simulink model "FCSMPC_IdealSDA"  (R2026a)
settings: Solver=FixedStepDiscrete  StopTime=inf  FixedStep=SimulinkTs
PreLoadFcn:
  | % Verzeichnis des Modells zum MATLAB-Pfad hinzufügen
  | modelDir = fileparts(get_param(bdroot, 'FileName'));
  | addpath(modelDir);
  | 
  | % Nur der Dateiname – kein Pfad!
  | set_param(bdroot, 'DataDictionary', 'FOC_params.sldd');
model workspace (MAT data in the model file):
  Np = Simulink.Parameter
  Np.Value = 5
  Np.Complexity = 'real'
  Np.Dimensions = [1 1]
  Np.DataType = 'double'
undefined symbols (not defined in the file or in its folder): dspblkCoreblockFVToolHelper, FCS, Filter, FOC, FOC_Control_Current_KIid, FOC_Control_Current_KIiq, FOC_Control_Current_KPid, FOC_Control_Current_KPiq, FOC_Control_Current_Krd, FOC_Control_Current_Krq, FOC_Control_Current_TclCur, FOC_Control_Current_Tnd, FOC_Control_Current_Tnq, FOC_Control_InverterVdc_V, FOC_Control_MotorImax_A, FOC_Control_MTPA_MTPV_nT_id_grid, FOC_Control_MTPA_MTPV_nT_iq_grid, FOC_Control_MTPA_MTPV_T_vec, FOC_Control_MTPA_MTPV_w_vec, FOC_Control_OpenLoop_Id_Ref_A, FOC_Control_OpenLoop_Iq_Ref_A, FOC_Control_OpenLoop_Ud_OpenLoop_V, FOC_Control_OpenLoop_Uq_OpenLoop_V, FOC_Control_RF_omegamech_rad_s, FOC_Control_RF_RateCurrent_A, FOC_Control_RF_RateTrq_Nm, FOC_Control_theta_mechOffsetFix, FOC_Control_theta_mechOffsetTime, FOC_Control_TorqueRef_Nm, FOC_Control_Umax_V, FOC_Flag_ClosedLoopControl, FOC_Flag_ControlStrategy, FOC_Flag_PWMEnable, FOC_Flag_ResetControl, FOC_Flag_TorqueControl, FOC_LUT_DQLimiter_DQ_LUTScaling, FOC_PWM_AZSPWMMethod, FOC_PWM_HybridMode, FOC_PWM_LB1, FOC_PWM_LB2, FOC_PWM_PWMManuel, FOC_PWM_RSPWMMethod, FOC_PWM_UB1, FOC_PWM_UB2, FOC_SampleTime_TsCur, gcbh, Plant, SimulinkTs
libraries: hdlsllib x2, autolibfluxpmsm x1, simulink x1
settings Model: DataDictionary=FOC_params.sldd  Creator=kara  LastModifiedBy=Cheng
settings DebuggingCC: ParameterPrecisionLossMsg=none
settings SimscapeCC: SimscapeNominalValues="[{\"value\":\"1\",\"unit\":\"A\"},{\"value\":\"1\",\"unit\":\"bar\"},{\"value\":\"1\",\"unit\":\"cm^2\"},{\"value\":\"1\",\"unit\":\"cm^3/s\"},{\"value\":\"1\",\"unit\":\"kJ/kg\"},{\"value\":\"1\",\"unit\":\"kW\"},{\"value\":\"1\",\"unit\":\"l\"},{\"value\":\"1\",\"unit\":\"N\"},{\"value\":\"1\",\"unit\":\"N*m\"},{\"value\":\"1\",\"unit\":\"V\"}]"  SimscapeLogType=none  SimscapeLogDataHistory=5000.0

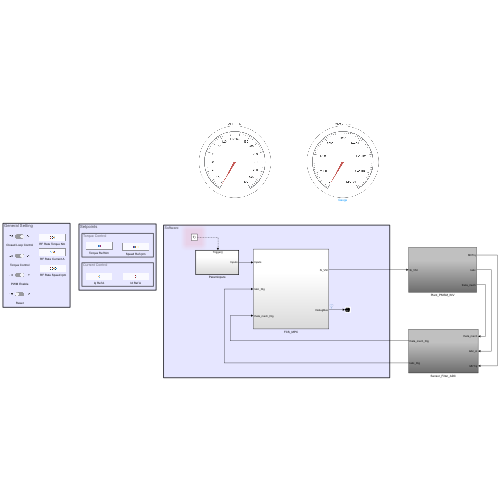
[thumbnail: Simulink's stored preview of the top-level diagram]
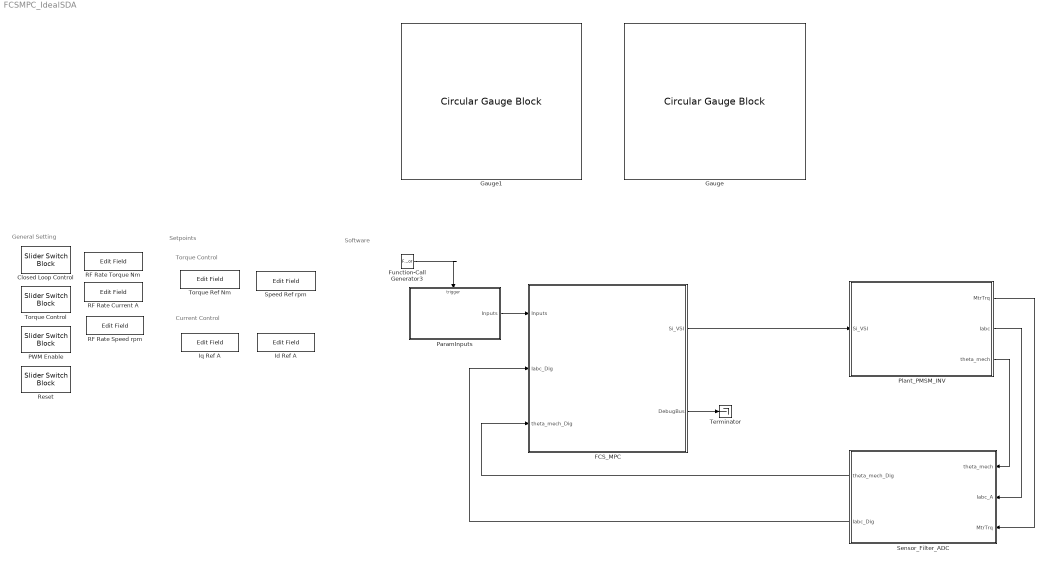
== system FCSMPC_IdealSDA ==
  note: Torque Control
  note: Software
  note: Current Control
  note: Setpoints
  note: General Setting
  Closed Loop Control : SliderSwitchBlock  LabelPosition=Hide
  FCS_MPC : Subsystem  VariantControl=AltPWM == 0
  Function-Call Generator3 : FunctionCallGenerator  SampleTime=FOC.SampleTime.TsSpeed
  Gauge : CircularGaugeBlock  ScaleMax=16000  FontColor=[0.0, 0.0, 0.0]
  Gauge1 : CircularGaugeBlock  ScaleMax=300  FontColor=[0.0, 0.0, 0.0]
  Id Ref A : EditField  LabelPosition=Hide  ShowInitialText=on  Alignment=Center
  Iq Ref A : EditField  LabelPosition=Hide  ShowInitialText=on  Alignment=Center
  PWM Enable : SliderSwitchBlock  LabelPosition=Hide
  ParamInputs : Subsystem
  Plant_PMSM_INV : Subsystem
  RF Rate Current A : EditField  LabelPosition=Hide  ShowInitialText=on  Alignment=Center
  RF Rate Speed rpm : EditField  LabelPosition=Hide  ShowInitialText=on  Alignment=Center
  RF Rate Torque Nm : EditField  LabelPosition=Hide  ShowInitialText=on  Alignment=Center
  Reset : SliderSwitchBlock  LabelPosition=Hide
  Sensor_Filter_ADC : Subsystem
  Speed Ref rpm : EditField  LabelPosition=Hide  ShowInitialText=on  Alignment=Center
  Terminator : Terminator
  Torque Control : SliderSwitchBlock  LabelPosition=Hide
  Torque Ref Nm : EditField  LabelPosition=Hide  ShowInitialText=on  Alignment=Center
  wires:
  ParamInputs/1(Inputs) -> FCS_MPC/1(Inputs)
  Function-Call Generator3/1 -> ParamInputs/Trigger
  Plant_PMSM_INV/2(Iabc) -> Sensor_Filter_ADC/2(Iabc_A)
  Plant_PMSM_INV/3(theta_mech) -> Sensor_Filter_ADC/1(theta_mech)
  FCS_MPC/1(Si_VSI) -> Plant_PMSM_INV/1(Si_VSI)
  Sensor_Filter_ADC/1(theta_mech_Dig) -> FCS_MPC/3(theta_mech_Dig)
  Plant_PMSM_INV/1(MtrTrq) -> Sensor_Filter_ADC/3(MtrTrq)
  Sensor_Filter_ADC/2(Iabc_Dig) -> FCS_MPC/2(Iabc_Dig)
  FCS_MPC/2(DebugBus) -> Terminator/1

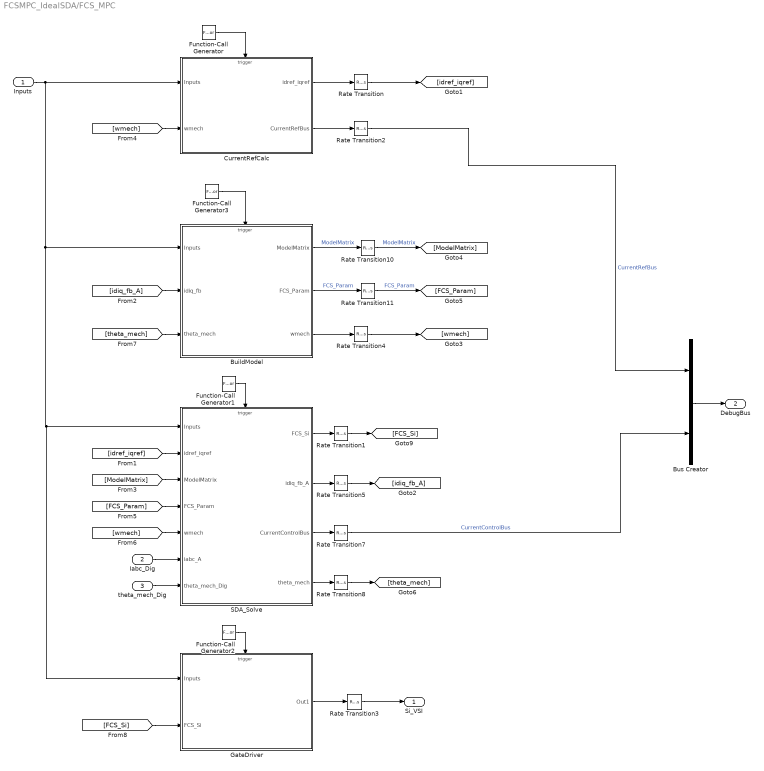
== system FCSMPC_IdealSDA/FCS_MPC ==
  Inputs : Inport
  Iabc_Dig : Inport  Port=2
  theta_mech_Dig : Inport  Port=3
  BuildModel : Subsystem
  Bus Creator : BusCreator  Inputs=2
  CurrentRefCalc : Subsystem
  Function-Call Generator : FunctionCallGenerator  SampleTime=FOC.SampleTime.TsSpeed
  Function-Call Generator1 : FunctionCallGenerator  SampleTime=FCS.Ts_SDA
  Function-Call Generator2 : FunctionCallGenerator  SampleTime=FOC.SampleTime.BSW.DeadTimeSample
  Function-Call Generator3 : FunctionCallGenerator  SampleTime=FCS.Ts_BuildModel
  GateDriver : Subsystem  TreatAsAtomicUnit=on
  Rate Transition{,1..5,7..8,10..11} (10 alike) : RateTransition  Deterministic=off
  SDA_Solve : Subsystem
  Si_VSI : Outport
  DebugBus : Outport  Port=2
  wires:
  Function-Call Generator/1 -> CurrentRefCalc/Trigger
  Function-Call Generator3/1 -> BuildModel/Trigger
  [wmech] -> CurrentRefCalc/2(wmech)
  CurrentRefCalc/1(idref_iqref) -> Rate Transition/1
  [idref_iqref] -> SDA_Solve/2(idref_iqref)
  Inputs/1 -> CurrentRefCalc/1(Inputs), GateDriver/1(Inputs), SDA_Solve/1(Inputs), BuildModel/1(Inputs)
  BuildModel/3(wmech) -> Rate Transition4/1
  CurrentRefCalc/2(CurrentRefBus) -> Rate Transition2/1
  Bus Creator/1 -> DebugBus/1
  Rate Transition/1 -> [idref_iqref]
  Rate Transition4/1 -> [wmech]
  Rate Transition2/1 -> Bus Creator/1  "CurrentRefBus"
  Rate Transition3/1 -> Si_VSI/1
  Function-Call Generator1/1 -> SDA_Solve/Trigger
  Iabc_Dig/1 -> SDA_Solve/6(iabc_A)
  SDA_Solve/2(idiq_fb_A) -> Rate Transition5/1
  Rate Transition5/1 -> [idiq_fb_A]
  [idiq_fb_A] -> BuildModel/2(idiq_fb)
  theta_mech_Dig/1 -> SDA_Solve/7(theta_mech_Dig)
  BuildModel/1(ModelMatrix) -> Rate Transition10/1  "ModelMatrix"
  BuildModel/2(FCS_Param) -> Rate Transition11/1  "FCS_Param"
  [ModelMatrix] -> SDA_Solve/3(ModelMatrix)
  [FCS_Param] -> SDA_Solve/4(FCS_Param)
  [wmech] -> SDA_Solve/5(wmech)
  SDA_Solve/3(CurrentControlBus) -> Rate Transition7/1
  Rate Transition7/1 -> Bus Creator/2  "CurrentControlBus"
  SDA_Solve/4(theta_mech) -> Rate Transition8/1
  Rate Transition8/1 -> [theta_mech]
  [theta_mech] -> BuildModel/3(theta_mech)
  Rate Transition11/1 -> [FCS_Param]  "FCS_Param"
  Rate Transition10/1 -> [ModelMatrix]  "ModelMatrix"
  Function-Call Generator2/1 -> GateDriver/Trigger
  GateDriver/1(Out1) -> Rate Transition3/1
  SDA_Solve/1(FCS_Si) -> Rate Transition1/1
  Rate Transition1/1 -> [FCS_Si]
  [FCS_Si] -> GateDriver/2(FCS_Si)

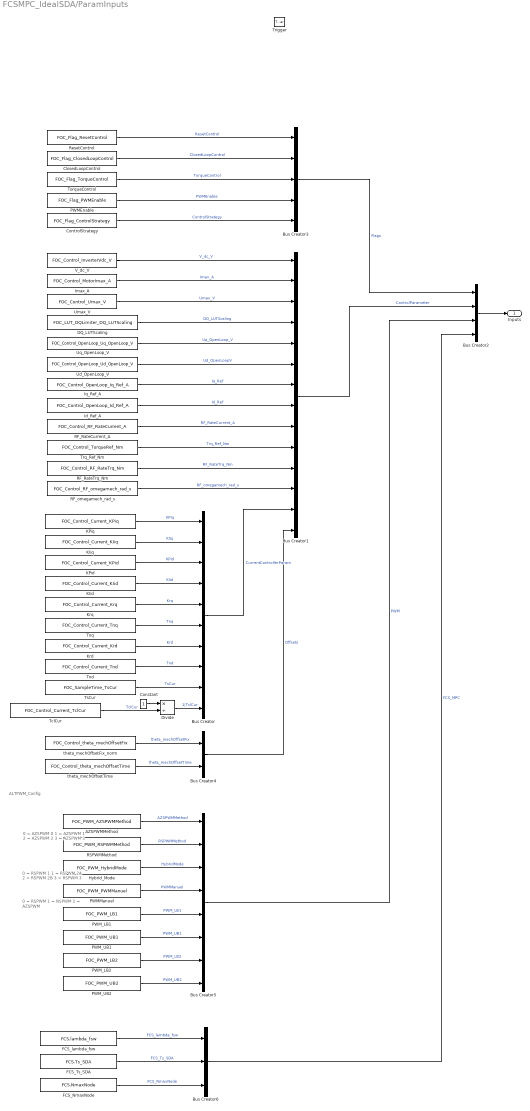
== system FCSMPC_IdealSDA/ParamInputs ==
  note: ALTPWM_Config
  note: 0 = RSPWM 1
      | 1 = RSPWM 2A
      | 2 = RSPWM 2B
      | 3 = RSPWM 3
  note: 0 = AZSPWM 0
      | 1 = AZSPWM 1
      | 2 = AZSPWM 2
      | 3 = AZSPWM 3
  note: 0 = RSPWM
      | 1 = NSPWM
      | 2 = AZSPWM
  Trigger : TriggerPort  TriggerType=function-call  VariantControl=(inherit)  SampleTimeType=periodic  SampleTime=FOC.SampleTime.TsSpeed  PortDimensions=1
  AZSPWMMethod : Constant  Value=FOC_PWM_AZSPWMMethod
  Bus Creator : BusCreator  Inputs=10
  Bus Creator1 : BusCreator  Inputs=14
  Bus Creator2 : BusCreator  Inputs=4
  Bus Creator3 : BusCreator  Inputs=5
  Bus Creator4 : BusCreator  Inputs=2
  Bus Creator5 : BusCreator  Inputs=8
  Bus Creator6 : BusCreator  Inputs=3
  ClosedLoopControl : Constant  Value=FOC_Flag_ClosedLoopControl
  Constant : Constant  OutDataTypeStr=SIScaling  SampleTime=-1
  ControlStrategy : Constant  Value=FOC_Flag_ControlStrategy
  DQ_LUTScaling : Constant  Value=FOC_LUT_DQLimiter_DQ_LUTScaling
  Divide : Product  Inputs=*/  OutDataTypeStr=SIScaling
  FCS_NmaxNode : Constant  Value=FCS.NmaxNode
  FCS_Ts_SDA : Constant  Value=FCS.Ts_SDA
  FCS_lambda_fsw : Constant  Value=FCS.lambda_fsw
  Hybrid_Mode : Constant  Value=FOC_PWM_HybridMode
  Id_Ref_A : Constant  Value=FOC_Control_OpenLoop_Id_Ref_A
  Imax_A : Constant  Value=FOC_Control_MotorImax_A
  Iq_Ref_A : Constant  Value=FOC_Control_OpenLoop_Iq_Ref_A
  KIid : Constant  Value=FOC_Control_Current_KIid
  KIiq : Constant  Value=FOC_Control_Current_KIiq
  KPid : Constant  Value=FOC_Control_Current_KPid
  KPiq : Constant  Value=FOC_Control_Current_KPiq
  Krd : Constant  Value=FOC_Control_Current_Krd
  Krq : Constant  Value=FOC_Control_Current_Krq
  PWMEnable : Constant  Value=FOC_Flag_PWMEnable
  PWMManuel : Constant  Value=FOC_PWM_PWMManuel
  PWM_LB1 : Constant  Value=FOC_PWM_LB1
  PWM_LB2 : Constant  Value=FOC_PWM_LB2
  PWM_UB1 : Constant  Value=FOC_PWM_UB1
  PWM_UB2 : Constant  Value=FOC_PWM_UB2
  RF_RateCurrent_A : Constant  Value=FOC_Control_RF_RateCurrent_A
  RF_RateTrq_Nm : Constant  Value=FOC_Control_RF_RateTrq_Nm
  RF_omegamech_rad_s : Constant  Value=FOC_Control_RF_omegamech_rad_s
  RSPWMMethod : Constant  Value=FOC_PWM_RSPWMMethod
  ResetControl : Constant  Value=FOC_Flag_ResetControl
  TclCur : Constant  Value=FOC_Control_Current_TclCur
  Tnd : Constant  Value=FOC_Control_Current_Tnd
  Tnq : Constant  Value=FOC_Control_Current_Tnq
  TorqueControl : Constant  Value=FOC_Flag_TorqueControl
  Trq_Ref_Nm : Constant  Value=FOC_Control_TorqueRef_Nm
  TsCur : Constant  Value=FOC_SampleTime_TsCur
  Ud_OpenLoop_V : Constant  Value=FOC_Control_OpenLoop_Ud_OpenLoop_V
  Umax_V : Constant  Value=FOC_Control_Umax_V
  Uq_OpenLoop_V : Constant  Value=FOC_Control_OpenLoop_Uq_OpenLoop_V
  V_dc_V : Constant  Value=FOC_Control_InverterVdc_V
  theta_mechOffsetFix_norm : Constant  Value=FOC_Control_theta_mechOffsetFix
  theta_mechOffsetTime : Constant  Value=FOC_Control_theta_mechOffsetTime
  Inputs : Outport
  wires:
  Bus Creator2/1 -> Inputs/1
  ClosedLoopControl/1 -> Bus Creator3/2  "ClosedLoopControl"
  TorqueControl/1 -> Bus Creator3/3  "TorqueControl"
  PWMEnable/1 -> Bus Creator3/4  "PWMEnable"
  Bus Creator3/1 -> Bus Creator2/1  "Flags"
  ResetControl/1 -> Bus Creator3/1  "ResetControl"
  ControlStrategy/1 -> Bus Creator3/5  "ControlStrategy"
  Ud_OpenLoop_V/1 -> Bus Creator1/6  "Ud_OpenLoopV"
  Uq_OpenLoop_V/1 -> Bus Creator1/5  "Uq_OpenLoop_V"
  DQ_LUTScaling/1 -> Bus Creator1/4  "DQ_LUTScaling"
  Umax_V/1 -> Bus Creator1/3  "Umax_V"
  Bus Creator1/1 -> Bus Creator2/2  "ControlParameter"
  Iq_Ref_A/1 -> Bus Creator1/7  "Iq_Ref"
  Id_Ref_A/1 -> Bus Creator1/8  "Id_Ref"
  Imax_A/1 -> Bus Creator1/2  "Imax_A"
  RF_RateTrq_Nm/1 -> Bus Creator1/11  "RF_RateTrq_Nm"
  Trq_Ref_Nm/1 -> Bus Creator1/10  "Trq_Ref_Nm"
  RF_RateCurrent_A/1 -> Bus Creator1/9  "RF_RateCurrent_A"
  Bus Creator/1 -> Bus Creator1/13  "CurrentControllerParam"
  V_dc_V/1 -> Bus Creator1/1  "V_dc_V"
  RF_omegamech_rad_s/1 -> Bus Creator1/12  "RF_omegamech_rad_s"
  theta_mechOffsetFix_norm/1 -> Bus Creator4/1  "theta_mechOffsetFix"
  theta_mechOffsetTime/1 -> Bus Creator4/2  "theta_mechOffsetTime"
  Bus Creator4/1 -> Bus Creator1/14  "Offsets"
  Bus Creator5/1 -> Bus Creator2/3  "PWM"
  PWM_UB1/1 -> Bus Creator5/6  "PWM_UB1"
  PWM_LB2/1 -> Bus Creator5/7  "PWM_LB2"
  AZSPWMMethod/1 -> Bus Creator5/1  "AZSPWMMethod"
  RSPWMMethod/1 -> Bus Creator5/2  "RSPWMMethod"
  PWM_LB1/1 -> Bus Creator5/5  "PWM_LB1"
  PWM_UB2/1 -> Bus Creator5/8  "PWM_UB2"
  Hybrid_Mode/1 -> Bus Creator5/3  "HybridMode"
  PWMManuel/1 -> Bus Creator5/4  "PWMManuel"
  TsCur/1 -> Bus Creator/9  "TsCur"
  KIiq/1 -> Bus Creator/2  "KIiq"
  Tnq/1 -> Bus Creator/6  "Tnq"
  Krd/1 -> Bus Creator/7  "Krd"
  KPid/1 -> Bus Creator/3  "KPid"
  Krq/1 -> Bus Creator/5  "Krq"
  Tnd/1 -> Bus Creator/8  "Tnd"
  KIid/1 -> Bus Creator/4  "KIid"
  KPiq/1 -> Bus Creator/1  "KPiq"
  TclCur/1 -> Divide/2  "TclCur"
  Divide/1 -> Bus Creator/10  "1|TclCur"
  Constant/1 -> Divide/1
  FCS_Ts_SDA/1 -> Bus Creator6/2  "FCS_Ts_SDA"
  FCS_lambda_fsw/1 -> Bus Creator6/1  "FCS_lambda_fsw"
  Bus Creator6/1 -> Bus Creator2/4  "FCS_MPC"
  FCS_NmaxNode/1 -> Bus Creator6/3  "FCS_NmaxNode"

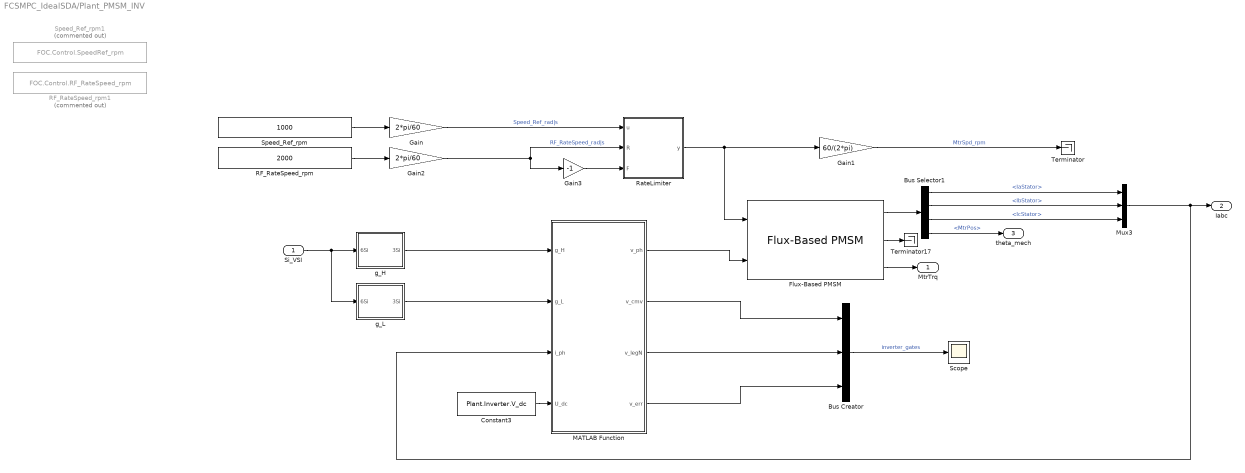
== system FCSMPC_IdealSDA/Plant_PMSM_INV ==
  Si_VSI : Inport
  Bus Creator : BusCreator  Inputs=3
  Bus Selector1 : BusSelector  OutputSignals=IaStator,IbStator,IcStator,MtrPos
  Constant3 : Constant  Value=Plant.Inverter.V_dc  SampleTime=-1
  Flux-Based PMSM : autolibfluxpmsm/Flux-Based PMSM  sim_type=Discrete  Ts=SimulinkTs  port_config=Speed  enable_hdl=off  flux_d=Plant.Fluxd_vec  n1=2  flux_q=Plant.Fluxq_vec  n2=2  id=Plant.FluxdFluxq_Id_grid'  iq=Plant.FluxdFluxq_Iq_grid'  preExtrapFlag=off  u1max=0.22457  u1min=-0.22607  u2max=0.42959  u2min=-0.4296  Rs=Plant.Motor.Rs  P=Plant.Motor.p  fluxdq0=[0 0]  theta_init=0  omega_init=0  mechanical=[0.0027, 4.924e-4, 0]  RefBlkName='autolibfluxpmsm/Flux-Based PMSM'  intPrec=23
      settings: LibrarySourceBlock=autolibemachines/Flux-Based PMSM
  Gain : Gain  Gain=2*pi/60
  Gain1 : Gain  Gain=60/(2*pi)
  Gain2 : Gain  Gain=2*pi/60
  Gain3 : Gain  Gain=-1
  MATLAB Function : MATLAB Function  TreatAsAtomicUnit=on
  Mux3 : Mux  Inputs=3
  RF_RateSpeed_rpm : Constant  Value=2000
  RF_RateSpeed_rpm1 : Constant  Commented=on  Value=FOC.Control.RF_RateSpeed_rpm
  RateLimiter : Stateflow chart  TreatAsAtomicUnit=on
  Scope : Scope
  Speed_Ref_rpm : Constant  Value=1000
  Speed_Ref_rpm1 : Constant  Commented=on  Value=FOC.Control.SpeedRef_rpm
  Terminator : Terminator
  Terminator17 : Terminator
  g_H : Subsystem
  g_L : Subsystem
  MtrTrq : Outport
  Iabc : Outport  Port=2
  theta_mech : Outport  Port=3
  wires:
  RateLimiter/1(y) -> Flux-Based PMSM/1, Gain1/1
  g_H/1(3Si) -> MATLAB Function/1(g_H)
  Bus Selector1/2 -> Mux3/2  "<IbStator>"
  Si_VSI/1 -> g_L/1(6Si), g_H/1(6Si)
  Bus Selector1/1 -> Mux3/1  "<IaStator>"
  Constant3/1 -> MATLAB Function/4(U_dc)
  Flux-Based PMSM/2 -> Terminator17/1
  Flux-Based PMSM/1 -> Bus Selector1/1
  Bus Selector1/3 -> Mux3/3  "<IcStator>"
  Gain1/1 -> Terminator/1  "MtrSpd_rpm"
  Flux-Based PMSM/3 -> MtrTrq/1
  Mux3/1 -> MATLAB Function/3(i_ph), Iabc/1
  Bus Selector1/4 -> theta_mech/1  "<MtrPos>"
  Gain3/1 -> RateLimiter/3(F)
  RF_RateSpeed_rpm/1 -> Gain2/1
  Speed_Ref_rpm/1 -> Gain/1
  Gain/1 -> RateLimiter/1(u)  "Speed_Ref_rad|s"
  Gain2/1 -> RateLimiter/2(R), Gain3/1  "RF_RateSpeed_rad|s"
  g_L/1(3Si) -> MATLAB Function/2(g_L)
  MATLAB Function/1(v_ph) -> Flux-Based PMSM/2
  MATLAB Function/2(v_cmv) -> Bus Creator/1
  MATLAB Function/4(v_err) -> Bus Creator/3
  MATLAB Function/3(v_legN) -> Bus Creator/2
  Bus Creator/1 -> Scope/1  "inverter_gates"

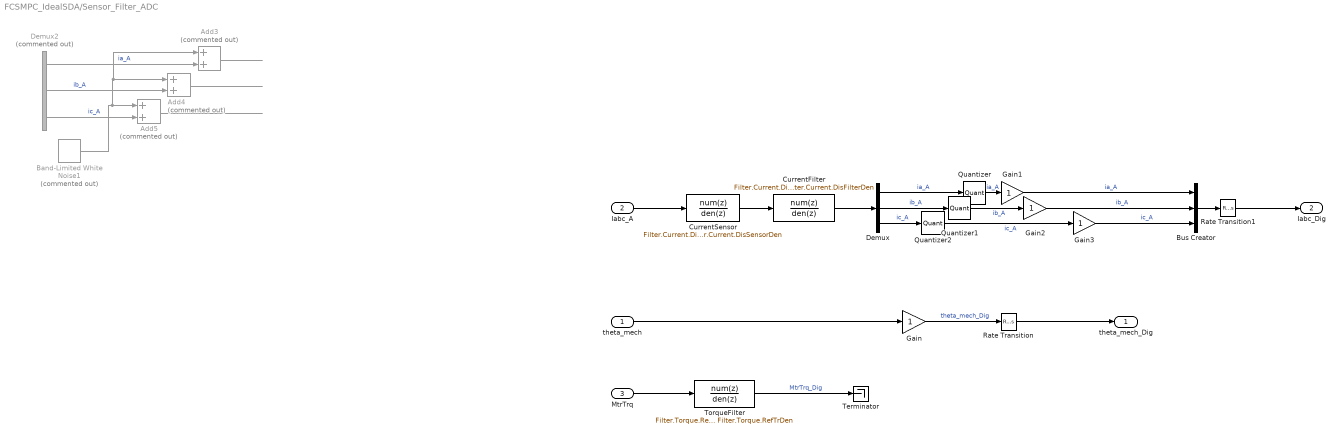
== system FCSMPC_IdealSDA/Sensor_Filter_ADC ==
  theta_mech : Inport
  Iabc_A : Inport  Port=2
  MtrTrq : Inport  Port=3
  Add3 : Sum  Commented=on
  Add4 : Sum  Commented=on
  Add5 : Sum  Commented=on
  Band-Limited White Noise1 : simulink/Sources/Band-Limited White Noise  Commented=on  Cov=[0.00001]  Ts=SimulinkTs  seed=[23341]
  Bus Creator : BusCreator  Inputs=3
  CurrentFilter : DiscreteTransferFcn  Numerator=Filter.Current.DisFilterNum  Denominator=Filter.Current.DisFilterDen
  CurrentSensor : DiscreteTransferFcn  LoadFcn=dspblkCoreblockFVToolHelper(gcbh,'load');  Numerator=Filter.Current.DisSensorNum  Denominator=Filter.Current.DisSensorDen
      settings: CopyFcn=dspblkCoreblockFVToolHelper(gcbh,'copy');  DeleteFcn=dspblkCoreblockFVToolHelper(gcbh,'close');  ModelCloseFcn=dspblkCoreblockFVToolHelper(gcbh,'close');  PreSaveFcn=dspblkCoreblockFVToolHelper(gcbh,'presave');  PostSaveFcn=dspblkCoreblockFVToolHelper(gcbh,'postsave');  CloseFcn=dspblkCoreblockFVToolHelper(gcbh,'close');
  Demux : Demux  Outputs=3
  Demux2 : Demux  Commented=on  Outputs=3
  Gain : Gain  OutDataTypeStr=HighScaling
  Gain1 : Gain  OutDataTypeStr=SIScaling
  Gain2 : Gain  OutDataTypeStr=SIScaling
  Gain3 : Gain  OutDataTypeStr=SIScaling
  Quantizer : Quantizer  QuantizationInterval=(10/32767)*264.04
  Quantizer1 : Quantizer  QuantizationInterval=(10/32767)*264.04
  Quantizer2 : Quantizer  QuantizationInterval=(10/32767)*264.04
  Rate Transition : RateTransition  Deterministic=off
  Rate Transition1 : RateTransition  Deterministic=off
  Terminator : Terminator
  TorqueFilter : DiscreteTransferFcn  Numerator=Filter.Torque.RefTrNum  Denominator=Filter.Torque.RefTrDen
  theta_mech_Dig : Outport
  Iabc_Dig : Outport  Port=2
  wires:
  MtrTrq/1 -> TorqueFilter/1
  CurrentSensor/1 -> CurrentFilter/1
  CurrentFilter/1 -> Demux/1
  TorqueFilter/1 -> Terminator/1  "MtrTrq_Dig"
  Demux/2 -> Quantizer1/1  "ib_A"
  Demux/3 -> Quantizer2/1  "ic_A"
  Demux/1 -> Quantizer/1  "ia_A"
  Bus Creator/1 -> Rate Transition1/1
  Gain/1 -> Rate Transition/1  "theta_mech_Dig"
  Gain1/1 -> Bus Creator/1  "ia_A"
  Gain2/1 -> Bus Creator/2  "ib_A"
  Gain3/1 -> Bus Creator/3  "ic_A"
  Rate Transition/1 -> theta_mech_Dig/1
  Rate Transition1/1 -> Iabc_Dig/1
  theta_mech/1 -> Gain/1
  Quantizer/1 -> Gain1/1  "ia_A"
  Quantizer1/1 -> Gain2/1  "ib_A"
  Quantizer2/1 -> Gain3/1  "ic_A"
  Iabc_A/1 -> CurrentSensor/1
  Demux2/1 -> Add3/2  "ia_A"
  Demux2/2 -> Add4/2  "ib_A"
  Demux2/3 -> Add5/2  "ic_A"
  Add5/1 -> ?
  Add4/1 -> ?
  Add3/1 -> ?
  ? -> Demux2/1
  Band-Limited White Noise1/1 -> Add5/1, Add4/1, Add3/1

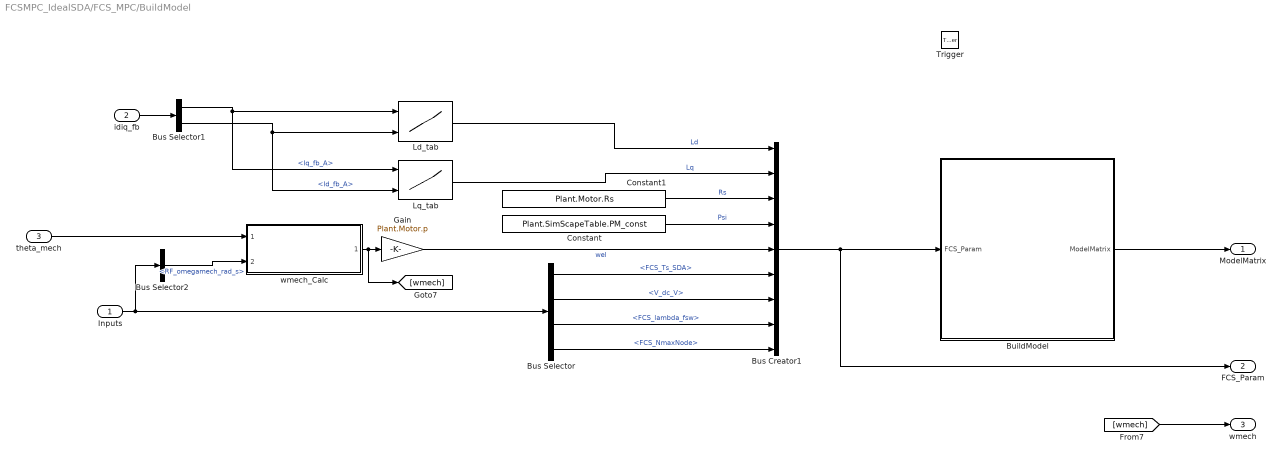
== system FCSMPC_IdealSDA/FCS_MPC/BuildModel ==
  Inputs : Inport
  idiq_fb : Inport  Port=2
  theta_mech : Inport  Port=3
  Trigger : TriggerPort  TriggerType=function-call  VariantControl=(inherit)  PropagateVarSize=Only when enabling  SampleTimeType=periodic  SampleTime=FCS.Ts_BuildModel  InitialTriggerSignalState=positive  PortDimensions=1
  BuildModel : Subsystem
  Bus Creator1 : BusCreator  Inputs=9
  Bus Selector : BusSelector  OutputSignals=FCS_MPC.FCS_Ts_SDA,ControlParameter.V_dc_V,FCS_MPC.FCS_lambda_fsw,FCS_MPC.FCS_NmaxNode
  Bus Selector1 : BusSelector  OutputSignals=Iq_fb_A,Id_fb_A
  Bus Selector2 : BusSelector  OutputSignals=ControlParameter.RF_omegamech_rad_s
  Constant : Constant  Value=Plant.SimScapeTable.PM_const  OutDataTypeStr=PWMGenSacling  SampleTime=-1
  Constant1 : Constant  Value=Plant.Motor.Rs  OutDataTypeStr=PWMGenSacling  SampleTime=-1
  Gain : Gain  Gain=Plant.Motor.p  OutDataTypeStr=RoughScaling
  Ld_tab : Lookup_n-D  BreakpointsForDimension1=Plant.SimScapeTable.iQ_vec  BreakpointsForDimension2=Plant.SimScapeTable.iD_vec  Table=Plant.SimScapeTable.Ld_tab'  ExtrapMethod=Clip  InternalRulePriority=Speed  RndMeth=Simplest
      settings: InputPortMap=u0,u1
  Lq_tab : Lookup_n-D  BreakpointsForDimension1=Plant.SimScapeTable.iQ_vec  BreakpointsForDimension2=Plant.SimScapeTable.iD_vec  Table=Plant.SimScapeTable.Lq_tab'  ExtrapMethod=Clip  InternalRulePriority=Speed  RndMeth=Simplest
      settings: InputPortMap=u0,u1
  wmech_Calc : Subsystem  ReferencedSubsystem=wmech_Calc
  ModelMatrix : Outport
  FCS_Param : Outport  Port=2
  wmech : Outport  Port=3
  wires:
  Ld_tab/1 -> Bus Creator1/1  "Ld"
  Lq_tab/1 -> Bus Creator1/2  "Lq"
  Constant/1 -> Bus Creator1/4  "Psi"
  Bus Selector/1 -> Bus Creator1/6  "<FCS_Ts_SDA>"
  Bus Selector/2 -> Bus Creator1/7  "<V_dc_V>"
  Bus Creator1/1 -> FCS_Param/1, BuildModel/1(FCS_Param)
  BuildModel/1(ModelMatrix) -> ModelMatrix/1
  Gain/1 -> Bus Creator1/5  "wel"
  Bus Selector/4 -> Bus Creator1/9  "<FCS_NmaxNode>"
  Bus Selector/3 -> Bus Creator1/8  "<FCS_lambda_fsw>"
  idiq_fb/1 -> Bus Selector1/1
  Bus Selector1/2 -> Lq_tab/2, Ld_tab/2  "<Id_fb_A>"
  Bus Selector1/1 -> Lq_tab/1, Ld_tab/1  "<Iq_fb_A>"
  Constant1/1 -> Bus Creator1/3  "Rs"
  theta_mech/1 -> wmech_Calc/1
  Bus Selector2/1 -> wmech_Calc/2  "<RF_omegamech_rad_s>"
  Inputs/1 -> Bus Selector/1, Bus Selector2/1
  [wmech] -> wmech/1
  wmech_Calc/1 -> [wmech], Gain/1

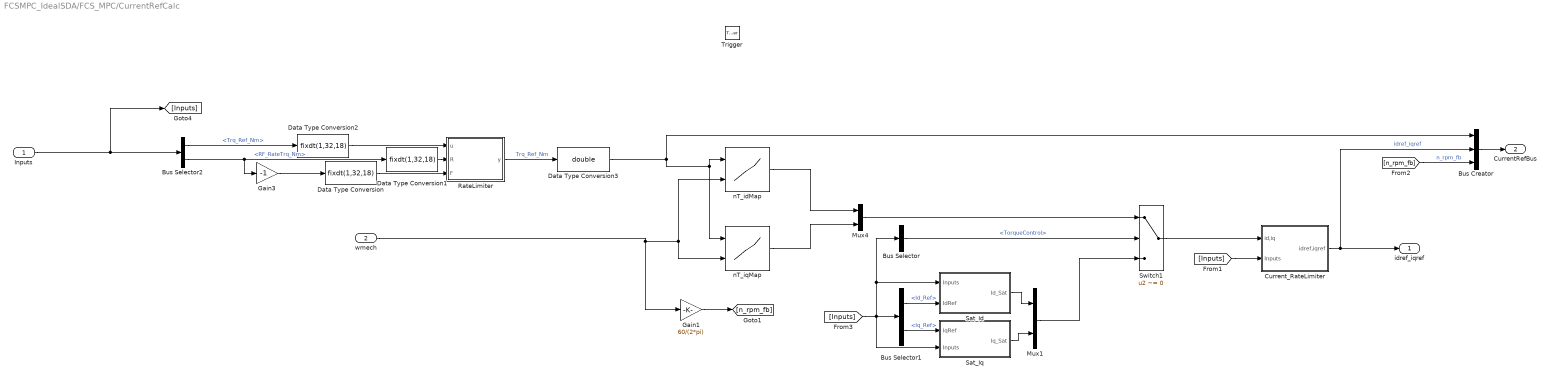
== system FCSMPC_IdealSDA/FCS_MPC/CurrentRefCalc ==
  Inputs : Inport
  wmech : Inport  Port=2
  Trigger : TriggerPort  TriggerType=function-call  VariantControl=(inherit)  PropagateVarSize=Only when enabling  SampleTimeType=periodic  SampleTime=FOC.SampleTime.TsSpeed  InitialTriggerSignalState=positive  PortDimensions=1
  Bus Creator : BusCreator  Inputs=3
  Bus Selector : BusSelector  OutputSignals=Flags.TorqueControl
  Bus Selector1 : BusSelector  OutputSignals=ControlParameter.Id_Ref,ControlParameter.Iq_Ref
  Bus Selector2 : BusSelector  OutputSignals=ControlParameter.Trq_Ref_Nm,ControlParameter.RF_RateTrq_Nm
  Current_RateLimiter : Subsystem
  Data Type Conversion : DataTypeConversion  OutDataTypeStr=fixdt(1,32,18)  SaturateOnIntegerOverflow=off  RndMeth=Floor
  Data Type Conversion1 : DataTypeConversion  OutDataTypeStr=fixdt(1,32,18)  SaturateOnIntegerOverflow=off  RndMeth=Floor
  Data Type Conversion2 : DataTypeConversion  OutDataTypeStr=fixdt(1,32,18)  SaturateOnIntegerOverflow=off  RndMeth=Floor
  Data Type Conversion3 : DataTypeConversion  OutDataTypeStr=double  SaturateOnIntegerOverflow=off  RndMeth=Floor
  Gain1 : Gain  Gain=60/(2*pi)  OutDataTypeStr=SIScaling
  Gain3 : Gain  Gain=-1  OutDataTypeStr=SIScaling
  Mux1 : Mux  Inputs=2
  Mux4 : Mux  Inputs=2
  RateLimiter : Stateflow chart  TreatAsAtomicUnit=on
  Sat_Id : Subsystem
  Sat_Iq : Subsystem
  Switch1 : Switch  Criteria=u2 ~= 0  OutDataTypeStr=SIScaling  SaturateOnIntegerOverflow=off  InputSameDT=off
  nT_idMap : Lookup_n-D  BreakpointsForDimension1=FOC_Control_MTPA_MTPV_T_vec  BreakpointsForDimension2=FOC_Control_MTPA_MTPV_w_vec  Table=FOC_Control_MTPA_MTPV_nT_id_grid  ExtrapMethod=Clip  InternalRulePriority=Speed  RndMeth=Simplest
      settings: InputPortMap=u0,u1
  nT_iqMap : Lookup_n-D  BreakpointsForDimension1=FOC_Control_MTPA_MTPV_T_vec  BreakpointsForDimension2=FOC_Control_MTPA_MTPV_w_vec  Table=FOC_Control_MTPA_MTPV_nT_iq_grid  ExtrapMethod=Clip  InternalRulePriority=Speed  RndMeth=Simplest
      settings: InputPortMap=u0,u1
  idref_iqref : Outport
  CurrentRefBus : Outport  Port=2
  wires:
  Bus Selector2/2 -> Data Type Conversion1/1, Gain3/1  "<RF_RateTrq_Nm>"
  Gain3/1 -> Data Type Conversion/1
  RateLimiter/1(y) -> Data Type Conversion3/1  "Trq_Ref_Nm"
  nT_iqMap/1 -> Mux4/2
  nT_idMap/1 -> Mux4/1
  Mux4/1 -> Switch1/1
  Bus Selector/1 -> Switch1/2  "<TorqueControl>"
  Bus Selector1/1 -> Sat_Id/2(IdRef)  "<Id_Ref>"
  Bus Selector1/2 -> Sat_Iq/1(IqRef)  "<Iq_Ref>"
  Mux1/1 -> Switch1/3
  Sat_Id/1(Id_Sat) -> Mux1/1
  Sat_Iq/1(Iq_Sat) -> Mux1/2
  Inputs/1 -> Bus Selector2/1, [Inputs]
  [Inputs] -> Sat_Iq/2(Inputs), Bus Selector/1, Sat_Id/1(Inputs), Bus Selector1/1
  Bus Selector2/1 -> Data Type Conversion2/1  "<Trq_Ref_Nm>"
  Switch1/1 -> Current_RateLimiter/1(id,iq)
  [Inputs] -> Current_RateLimiter/2(Inputs)
  Current_RateLimiter/1(idref,iqref) -> idref_iqref/1, Bus Creator/2  "idref_iqref"
  Bus Creator/1 -> CurrentRefBus/1
  [n_rpm_fb] -> Bus Creator/3  "n_rpm_fb"
  wmech/1 -> Gain1/1, nT_iqMap/2, nT_idMap/2
  Gain1/1 -> [n_rpm_fb]
  Data Type Conversion/1 -> RateLimiter/3(F)
  Data Type Conversion1/1 -> RateLimiter/2(R)
  Data Type Conversion2/1 -> RateLimiter/1(u)
  Data Type Conversion3/1 -> nT_iqMap/1, nT_idMap/1, Bus Creator/1

== system FCSMPC_IdealSDA/FCS_MPC/GateDriver ==
  Inputs : Inport
  FCS_Si : Inport  Port=2
  Trigger : TriggerPort  TriggerType=function-call  VariantControl=(inherit)  SampleTimeType=periodic  SampleTime=FOC.SampleTime.BSW.DeadTimeSample
  Bus Selector : BusSelector  OutputSignals=Flags.PWMEnable
  Constant4 : Constant  Value=[0 0 0 0 0 0]  OutDataTypeStr=uint8  SampleTime=-1
  GateDriver : Subsystem  ReferencedSubsystem=GateDriver  DeadTime=FOC.SampleTime.BSW.DeadTime  DeadTimeSample=FOC.SampleTime.BSW.DeadTimeSample
  Switch1 : Switch  Criteria=u2 ~= 0  SaturateOnIntegerOverflow=off  InputSameDT=off
  Out1 : Outport
  wires:
  FCS_Si/1 -> GateDriver/1
  GateDriver/1 -> Switch1/1
  Constant4/1 -> Switch1/3
  Switch1/1 -> Out1/1
  Inputs/1 -> Bus Selector/1
  Bus Selector/1 -> Switch1/2  "<PWMEnable>"

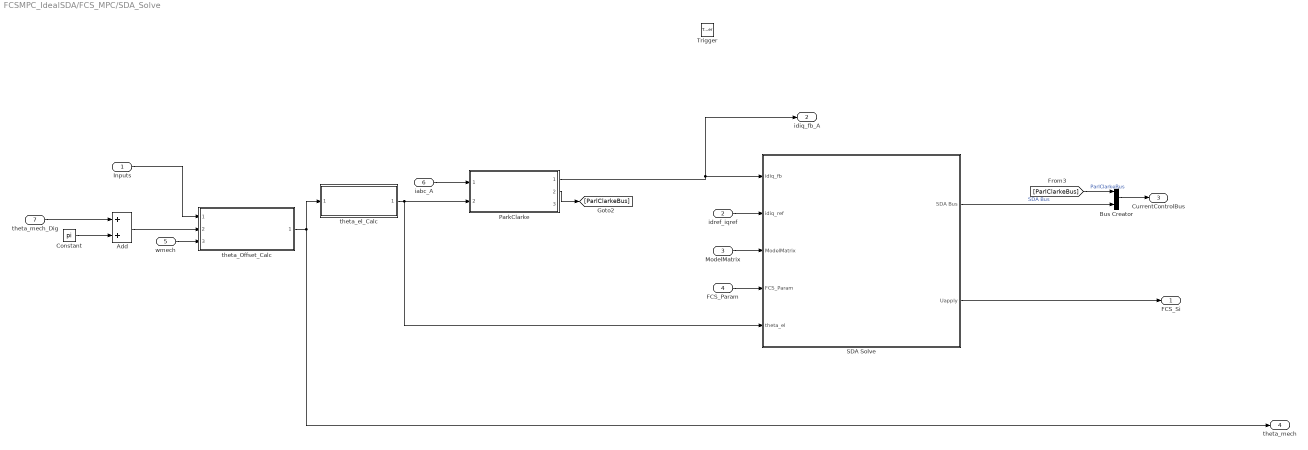
== system FCSMPC_IdealSDA/FCS_MPC/SDA_Solve ==
  Inputs : Inport
  idref_iqref : Inport  Port=2
  ModelMatrix : Inport  Port=3
  FCS_Param : Inport  Port=4
  wmech : Inport  Port=5
  iabc_A : Inport  Port=6
  theta_mech_Dig : Inport  Port=7
  Trigger : TriggerPort  TriggerType=function-call  VariantControl=(inherit)  PropagateVarSize=Only when enabling  SampleTimeType=periodic  SampleTime=FCS.Ts_SDA  InitialTriggerSignalState=positive  PortDimensions=1
  Add : Sum  OutDataTypeStr=HighScaling
  Bus Creator : BusCreator  Inputs=2
  Constant : Constant  Value=pi  OutDataTypeStr=HighScaling
  ParkClarke : Subsystem  ReferencedSubsystem=ParkClarke
  SDA Solve : Subsystem
  theta_Offset_Calc : Subsystem  ReferencedSubsystem=theta_Offset_Calc
  theta_el_Calc : Subsystem  ReferencedSubsystem=theta_el_Calc
  FCS_Si : Outport
  idiq_fb_A : Outport  Port=2
  CurrentControlBus : Outport  Port=3
  theta_mech : Outport  Port=4
  wires:
  SDA Solve/1(SDA Bus) -> Bus Creator/2  "SDA Bus"
  ModelMatrix/1 -> SDA Solve/3(ModelMatrix)
  ParkClarke/1 -> idiq_fb_A/1, SDA Solve/1(idiq_fb)
  idref_iqref/1 -> SDA Solve/2(idiq_ref)
  wmech/1 -> theta_Offset_Calc/3
  theta_Offset_Calc/1 -> theta_mech/1, theta_el_Calc/1
  ParkClarke/2 -> [ParlClarkeBus]
  Inputs/1 -> theta_Offset_Calc/1
  theta_el_Calc/1 -> SDA Solve/5(theta_el), ParkClarke/2
  iabc_A/1 -> ParkClarke/1
  Add/1 -> theta_Offset_Calc/2
  theta_mech_Dig/1 -> Add/1
  Constant/1 -> Add/2
  FCS_Param/1 -> SDA Solve/4(FCS_Param)
  [ParlClarkeBus] -> Bus Creator/1  "ParlClarkeBus"
  Bus Creator/1 -> CurrentControlBus/1
  SDA Solve/2(Uapply) -> FCS_Si/1

== system FCSMPC_IdealSDA/Plant_PMSM_INV/g_H ==
  6Si : Inport
  Demux2 : Demux  Outputs=6
  Mux2 : Mux  Inputs=3
  Terminator12 : Terminator
  Terminator13 : Terminator
  Terminator14 : Terminator
  3Si : Outport
  wires:
  Demux2/1 -> Mux2/1
  Demux2/3 -> Mux2/2
  Demux2/2 -> Terminator12/1
  Demux2/4 -> Terminator13/1
  Demux2/5 -> Mux2/3
  Demux2/6 -> Terminator14/1
  Mux2/1 -> 3Si/1
  6Si/1 -> Demux2/1

== system FCSMPC_IdealSDA/Plant_PMSM_INV/g_L ==
  6Si : Inport
  Demux2 : Demux  Outputs=6
  Mux2 : Mux  Inputs=3
  Terminator1 : Terminator
  Terminator13 : Terminator
  Terminator14 : Terminator
  3Si : Outport
  wires:
  6Si/1 -> Demux2/1
  Mux2/1 -> 3Si/1
  Demux2/6 -> Mux2/3
  Demux2/5 -> Terminator14/1
  Demux2/4 -> Mux2/2
  Demux2/2 -> Mux2/1
  Demux2/3 -> Terminator13/1
  Demux2/1 -> Terminator1/1

== system FCSMPC_IdealSDA/FCS_MPC/BuildModel/BuildModel ==
  FCS_Param : Inport
  Build_Model : MATLAB Function  TreatAsAtomicUnit=on
  Bus Creator2 : BusCreator  Inputs=9
  Bus Selector1 : BusSelector  OutputSignals=V_dc_V,FCS_lambda_fsw
  Bus Selector2 : BusSelector  OutputSignals=Ld,Lq,Rs,Psi,wel,FCS_Ts_SDA
  Discretize_PMSM : MATLAB Function  TreatAsAtomicUnit=on
  ModelMatrix : Outport
  wires:
  Discretize_PMSM/3(fd) -> Build_Model/2(fd), Bus Creator2/3  "fd"
  Discretize_PMSM/2(Ad) -> Build_Model/1(Ad), Bus Creator2/2  "Ad"
  Bus Selector1/2 -> Build_Model/4(lambda_fsw)  "<FCS_lambda_fsw>"
  Bus Creator2/1 -> ModelMatrix/1
  Discretize_PMSM/1(Bd) -> Bus Creator2/1  "Bd"
  FCS_Param/1 -> Bus Selector2/1, Bus Selector1/1
  Build_Model/4(Lambdafsw_SE) -> Bus Creator2/7  "Lambdafsw_SE"
  Build_Model/2(Phi) -> Bus Creator2/5  "Phi"
  Build_Model/3(Lambdafsw_Ssquare) -> Bus Creator2/6  "Lambdafsw_Ssquare"
  Build_Model/1(Gamma) -> Bus Creator2/4  "Gamma"
  Bus Selector1/1 -> Build_Model/3(Vdc)  "<V_dc_V>"
  Bus Selector2/1 -> Discretize_PMSM/1(Ld)  "<Ld>"
  Bus Selector2/2 -> Discretize_PMSM/2(Lq)  "<Lq>"
  Bus Selector2/3 -> Discretize_PMSM/3(Rs)  "<Rs>"
  Bus Selector2/4 -> Discretize_PMSM/4(Psi)  "<Psi>"
  Bus Selector2/6 -> Discretize_PMSM/6(Ts)  "<FCS_Ts_SDA>"
  Bus Selector2/5 -> Discretize_PMSM/5(wel)  "<wel>"
  Build_Model/5(Apow) -> Bus Creator2/8  "Apow"
  Build_Model/6(Bs_TI) -> Bus Creator2/9  "Bs_TI"

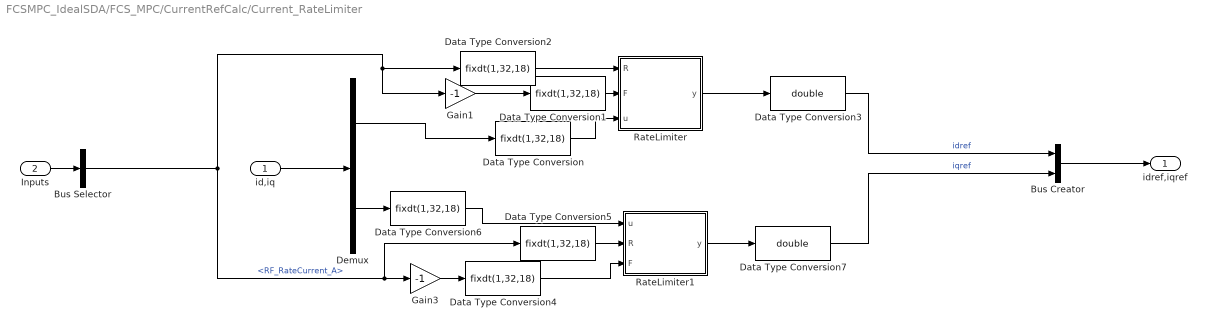
== system FCSMPC_IdealSDA/FCS_MPC/CurrentRefCalc/Current_RateLimiter ==
  id,iq : Inport
  Inputs : Inport  Port=2
  Bus Creator : BusCreator  Inputs=2
  Bus Selector : BusSelector  OutputSignals=ControlParameter.RF_RateCurrent_A
  Data Type Conversion{,1..2,4..6} (6 alike) : DataTypeConversion  OutDataTypeStr=fixdt(1,32,18)  SaturateOnIntegerOverflow=off  RndMeth=Floor
  Data Type Conversion3 : DataTypeConversion  OutDataTypeStr=double  SaturateOnIntegerOverflow=off  RndMeth=Floor
  Data Type Conversion7 : DataTypeConversion  OutDataTypeStr=double  SaturateOnIntegerOverflow=off  RndMeth=Floor
  Demux : Demux  Outputs=2
  Gain1 : Gain  Gain=-1  OutDataTypeStr=SIScaling
  Gain3 : Gain  Gain=-1  OutDataTypeStr=SIScaling
  RateLimiter : Stateflow chart  TreatAsAtomicUnit=on
      settings: PortSchema="{\"entries\":[{\"content\":{\"sides\":[{\"content\":{\"connectorIds\":[\"In2\",\"In3\",\"In1\"]},\"type\":\"ConnectorPlacement.EquallySpacedRectSide\",\"uuid\":\"9e69b296-78c9-4fde-bd06-f4cd15a9dc30\"},{\"content\":{\"connectorIds\":[\"Out1\"],\"side\":\"RIGHT\"},\"type\":\"ConnectorPlacement.EquallySpacedRectSide\",\"uuid\":\"c0eff11d-c292-417c-b924-d71f0425fe2c\"},{\"content\":{\"side\":\"TOP\"},\"type\":\"ConnectorPlacement.EquallySpacedRectSide\",\"uuid\":\"8270ba85-b05e-4504-bf71-02f9e02e7911\"}]},\"type\":\"ConnectorPlacement.EquallySpacedConnector\",\"uuid\":\"a73bdb84-3094-4ea9-abb8-664d745b6493\"}],\"packageUris\":[\"http://schema.mathworks.com/mf0/Connector/R2020b\"],\"version\":\"1.0\"}"
  RateLimiter1 : Stateflow chart  TreatAsAtomicUnit=on
  idref,iqref : Outport
  wires:
  RateLimiter/1(y) -> Data Type Conversion3/1
  id,iq/1 -> Demux/1
  Bus Creator/1 -> idref,iqref/1
  Demux/2 -> Data Type Conversion6/1
  Inputs/1 -> Bus Selector/1
  Bus Selector/1 -> Gain1/1, Data Type Conversion2/1, Data Type Conversion5/1, Gain3/1  "<RF_RateCurrent_A>"
  Gain3/1 -> Data Type Conversion4/1
  RateLimiter1/1(y) -> Data Type Conversion7/1
  Gain1/1 -> Data Type Conversion1/1
  Demux/1 -> Data Type Conversion/1
  Data Type Conversion2/1 -> RateLimiter/2(R)
  Data Type Conversion3/1 -> Bus Creator/1  "idref"
  Data Type Conversion1/1 -> RateLimiter/3(F)
  Data Type Conversion/1 -> RateLimiter/1(u)
  Data Type Conversion6/1 -> RateLimiter1/1(u)
  Data Type Conversion5/1 -> RateLimiter1/2(R)
  Data Type Conversion4/1 -> RateLimiter1/3(F)
  Data Type Conversion7/1 -> Bus Creator/2  "iqref"

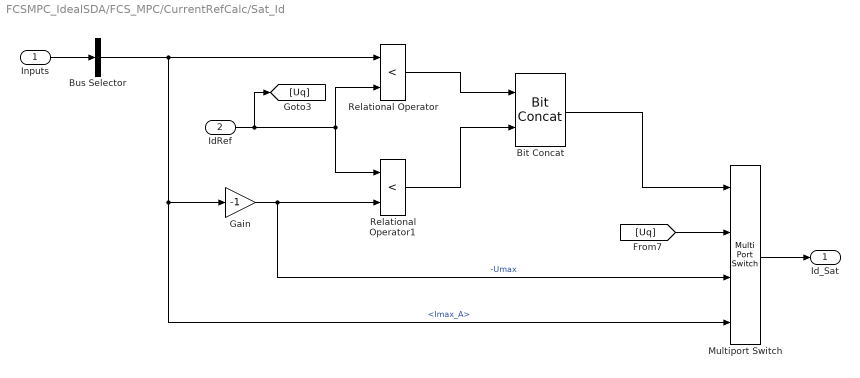
== system FCSMPC_IdealSDA/FCS_MPC/CurrentRefCalc/Sat_Id ==
  Inputs : Inport
  IdRef : Inport  Port=2
  Bit Concat : hdlsllib/Logic and Bit Operations/Bit Concat  numInputs=2
  Bus Selector : BusSelector  OutputSignals=ControlParameter.Imax_A
  Gain : Gain  Gain=-1  OutDataTypeStr=SIScaling
  Multiport Switch : MultiPortSwitch  DataPortOrder=Zero-based contiguous  zeroidx=on  OutDataTypeStr=SIScaling  SaturateOnIntegerOverflow=off  InputSameDT=off
  Relational Operator : RelationalOperator  Operator=<  OutDataTypeStr=boolean  RndMeth=Simplest  InputSameDT=off
  Relational Operator1 : RelationalOperator  Operator=<  OutDataTypeStr=boolean  RndMeth=Simplest  InputSameDT=off
  Id_Sat : Outport
  wires:
  IdRef/1 -> Relational Operator/2, Relational Operator1/1, [Uq]
  Gain/1 -> Multiport Switch/3, Relational Operator1/2  "-Umax"
  Relational Operator/1 -> Bit Concat/1
  Relational Operator1/1 -> Bit Concat/2
  Bit Concat/1 -> Multiport Switch/1
  Multiport Switch/1 -> Id_Sat/1
  [Uq] -> Multiport Switch/2
  Bus Selector/1 -> Multiport Switch/4, Gain/1, Relational Operator/1  "<Imax_A>"
  Inputs/1 -> Bus Selector/1

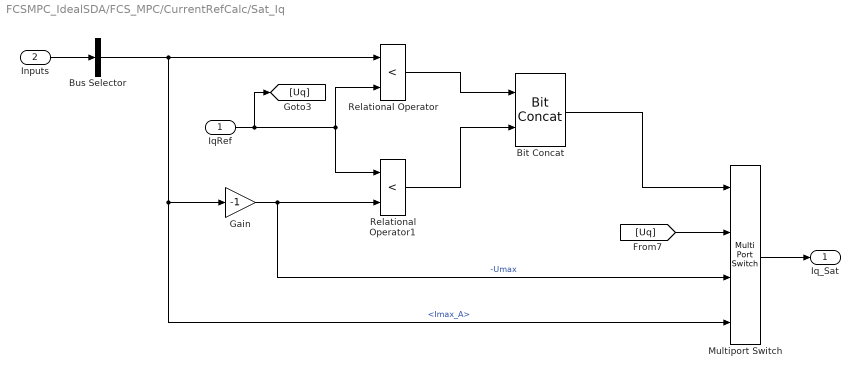
== system FCSMPC_IdealSDA/FCS_MPC/CurrentRefCalc/Sat_Iq ==
  IqRef : Inport
  Inputs : Inport  Port=2
  Bit Concat : hdlsllib/Logic and Bit Operations/Bit Concat  numInputs=2
  Bus Selector : BusSelector  OutputSignals=ControlParameter.Imax_A
  Gain : Gain  Gain=-1  OutDataTypeStr=SIScaling
  Multiport Switch : MultiPortSwitch  DataPortOrder=Zero-based contiguous  zeroidx=on  OutDataTypeStr=SIScaling  SaturateOnIntegerOverflow=off  InputSameDT=off
  Relational Operator : RelationalOperator  Operator=<  OutDataTypeStr=boolean  RndMeth=Simplest  InputSameDT=off
  Relational Operator1 : RelationalOperator  Operator=<  OutDataTypeStr=boolean  RndMeth=Simplest  InputSameDT=off
  Iq_Sat : Outport
  wires:
  Inputs/1 -> Bus Selector/1
  Bus Selector/1 -> Relational Operator/1, Gain/1, Multiport Switch/4  "<Imax_A>"
  [Uq] -> Multiport Switch/2
  Multiport Switch/1 -> Iq_Sat/1
  Bit Concat/1 -> Multiport Switch/1
  Relational Operator1/1 -> Bit Concat/2
  Relational Operator/1 -> Bit Concat/1
  Gain/1 -> Relational Operator1/2, Multiport Switch/3  "-Umax"
  IqRef/1 -> [Uq], Relational Operator1/1, Relational Operator/2

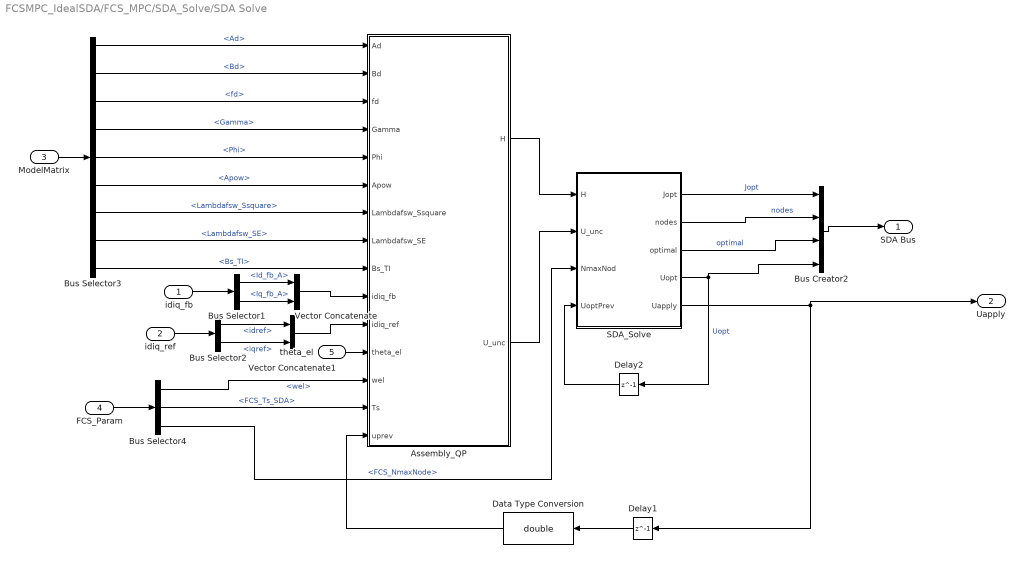
== system FCSMPC_IdealSDA/FCS_MPC/SDA_Solve/SDA Solve ==
  idiq_fb : Inport
  idiq_ref : Inport  Port=2
  ModelMatrix : Inport  Port=3
  FCS_Param : Inport  Port=4
  theta_el : Inport  Port=5
  Assembly_QP : MATLAB Function  TreatAsAtomicUnit=on
  Bus Creator2 : BusCreator  Inputs=4
  Bus Selector1 : BusSelector  OutputSignals=Id_fb_A,Iq_fb_A
  Bus Selector2 : BusSelector  OutputSignals=idref,iqref
  Bus Selector3 : BusSelector  OutputSignals=Ad,Bd,fd,Gamma,Phi,Apow,Lambdafsw_Ssquare,Lambdafsw_SE,Bs_TI
  Bus Selector4 : BusSelector  OutputSignals=wel,FCS_Ts_SDA,FCS_NmaxNode
  Data Type Conversion : DataTypeConversion  OutDataTypeStr=double  SaturateOnIntegerOverflow=off  RndMeth=Floor
  Delay1 : Delay  DelayLength=1  InitialCondition=zeros(3,1)
  Delay2 : Delay  DelayLength=1  InitialCondition=zeros(15,1)
  SDA_Solve : MATLAB Function  TreatAsAtomicUnit=on
  Vector Concatenate : Concatenate
  Vector Concatenate1 : Concatenate
  SDA Bus : Outport
  Uapply : Outport  Port=2
  wires:
  Bus Selector3/3 -> Assembly_QP/3(fd)  "<fd>"
  Bus Selector3/1 -> Assembly_QP/1(Ad)  "<Ad>"
  Assembly_QP/1(H) -> SDA_Solve/1(H)
  Bus Selector4/2 -> Assembly_QP/14(Ts)  "<FCS_Ts_SDA>"
  Bus Selector4/1 -> Assembly_QP/13(wel)  "<wel>"
  Bus Selector4/3 -> SDA_Solve/3(NmaxNod)  "<FCS_NmaxNode>"
  Bus Selector3/9 -> Assembly_QP/9(Bs_TI)  "<Bs_TI>"
  Bus Selector3/6 -> Assembly_QP/6(Apow)  "<Apow>"
  Bus Selector3/8 -> Assembly_QP/8(Lambdafsw_SE)  "<Lambdafsw_SE>"
  Bus Selector3/7 -> Assembly_QP/7(Lambdafsw_Ssquare)  "<Lambdafsw_Ssquare>"
  Bus Selector3/5 -> Assembly_QP/5(Phi)  "<Phi>"
  Bus Selector3/4 -> Assembly_QP/4(Gamma)  "<Gamma>"
  Bus Selector3/2 -> Assembly_QP/2(Bd)  "<Bd>"
  ModelMatrix/1 -> Bus Selector3/1
  SDA_Solve/3(optimal) -> Bus Creator2/3  "optimal"
  Delay1/1 -> Data Type Conversion/1
  idiq_fb/1 -> Bus Selector1/1
  Bus Selector2/1 -> Vector Concatenate1/1  "<idref>"
  Bus Selector1/2 -> Vector Concatenate/2  "<Iq_fb_A>"
  Vector Concatenate1/1 -> Assembly_QP/11(idiq_ref)
  Bus Selector2/2 -> Vector Concatenate1/2  "<iqref>"
  FCS_Param/1 -> Bus Selector4/1
  SDA_Solve/4(Uopt) -> Bus Creator2/4, Delay2/1  "Uopt"
  Assembly_QP/2(U_unc) -> SDA_Solve/2(U_unc)
  SDA_Solve/1(Jopt) -> Bus Creator2/1  "Jopt"
  Bus Selector1/1 -> Vector Concatenate/1  "<Id_fb_A>"
  SDA_Solve/2(nodes) -> Bus Creator2/2  "nodes"
  idiq_ref/1 -> Bus Selector2/1
  Bus Creator2/1 -> SDA Bus/1
  Vector Concatenate/1 -> Assembly_QP/10(idiq_fb)
  theta_el/1 -> Assembly_QP/12(theta_el)
  Data Type Conversion/1 -> Assembly_QP/15(uprev)
  SDA_Solve/5(Uapply) -> Uapply/1, Delay1/1
  Delay2/1 -> SDA_Solve/4(UoptPrev)

== matlab function FCSMPC_IdealSDA/Plant_PMSM_INV/MATLAB Function ==
  data: g_H input; g_L input; v_ph output; i_ph input; U_dc input; v_cmv output; v_legN output; v_err output
function [v_ph, v_cmv, v_legN, v_err] = inverter_model_gates(g_H, g_L, i_ph, U_dc)
%#codegen
% INVERTER_MODEL_GATES  Zweistufiger B6-Wechselrichter, zustandslos.
%
%   Erwartet die sechs Gate-Signale, in denen die Totzeit bereits
%   enthalten ist (waehrend der Totzeit sind g_H(k) und g_L(k) beide 0).
%   Dadurch benoetigt der Block keinen internen Zaehler und keine
%   Rueckfuehrung -- er ist rein kombinatorisch.
%
%   Eingaenge:
%     g_H   3x1 logical  Gate oberer Schalter je Bein
%     g_L   3x1 logical  Gate unterer Schalter je Bein
%     i_ph  3x1 double   Phasenstroeme [A], Zaehlpfeil aus dem Bein heraus
%     U_dc  1x1 double   Zwischenkreisspannung [V]
%
%   Ausgaenge:
%     v_ph   3x1 double  Strangspannungen gegen Sternpunkt [V]
%     v_cmv  1x1 double  Gleichtaktspannung gegen DC-Mittelpunkt [V]
%     v_legN 3x1 double  Beinpotenziale gegen DC-Minus [V]
%     v_err  3x1 double  Abweichung vom idealen Kommandowert [V] (Diagnose)

% ------------------------------------------------------------------
% Parameter
% ------------------------------------------------------------------
U_CE = 1.5;    % IGBT-Durchlassspannung [V]  (0 -> idealer Schalter)
U_F  = 1.2;    % Diodenflussspannung [V]     (0 -> ideale Diode)

v_legN    = zeros(3,1);
v_leg_cmd = zeros(3,1);

for k = 1:3

    ik = i_ph(k);
    hi = g_H(k);
    lo = g_L(k);

    if hi && ~lo
        % ===== Oberer Schalter eingeschaltet =====
        if ik >= 0
            v_legN(k) = U_dc - U_CE;    % oberer IGBT leitet
        else
            v_legN(k) = U_dc + U_F;     % obere Diode leitet
        end
        v_leg_cmd(k) = U_dc;

    elseif ~hi && lo
        % ===== Unterer Schalter eingeschaltet =====
        if ik > 0
            v_legN(k) = -U_F;           % untere Diode leitet
        else
            v_legN(k) = U_CE;           % unterer IGBT leitet
        end
        v_leg_cmd(k) = 0;

    elseif ~hi && ~lo
        % ===== TOTZEIT: beide Gates aus, Diode entscheidet =====
        if ik > 0
            v_legN(k) = -U_F;           % untere Freilaufdiode
            v_leg_cmd(k) = 0;
        else
            v_legN(k) = U_dc + U_F;     % obere Freilaufdiode
            v_leg_cmd(k) = U_dc;
        end

    else
        % ===== Beide Gates an: Bruecken-Kurzschluss =====
        % Physikalisch ein Fehlerfall. Hier als halbe Zwischenkreis-
        % spannung modelliert, damit die Simulation nicht divergiert.
        v_legN(k)    = 0.5 * U_dc;
        v_leg_cmd(k) = 0.5 * U_dc;
    end
end

% ------------------------------------------------------------------
% Sternpunktpotenzial, Strangspannungen, Gleichtaktspannung
% ------------------------------------------------------------------
% Symmetrische Last mit isoliertem Sternpunkt: Summe der Strangspannungen
% ist null, daraus folgt v_nN als Mittelwert der Beinpotenziale.
v_nN  = (v_legN(1) + v_legN(2) + v_legN(3)) / 3;

v_ph  = v_legN - v_nN;              % treiben die Maschine
v_cmv = v_nN - 0.5 * U_dc;          % gegen DC-Mittelpunkt

v_err = v_legN - v_leg_cmd;         % Diagnose: Abweichung vom Ideal

end

== matlab function FCSMPC_IdealSDA/FCS_MPC/BuildModel/BuildModel/Build_Model ==
  data: Ad input; fd input; Gamma output size=[2*Np 2]; Phi output size=[2*Np 1]; Lambdafsw_Ssquare output size=[3*Np 3*Np]; Lambdafsw_SE output size=[3*Np 3]; Apow output size=[2*(Np+1) 2]; Bs_TI output size=[2 3]; Vdc input; lambda_fsw input
function [Gamma, Phi, Lambdafsw_Ssquare, Lambdafsw_SE, Apow, Bs_TI]    = BuildModel(Ad, fd, Vdc, lambda_fsw)
Np = 5;
nu = 3;  ny = 2;
C  = eye(ny);
Apow = zeros(ny*(Np+1), ny);
Apow(1:ny, :) = eye(ny);
for m = 1:Np
    Apow(m*ny + (1:ny), :) = Apow((m-1)*ny + (1:ny), :) * Ad;
end
Bs_TI = switch_to_alphabeta(Vdc);

Gamma = zeros(ny*Np, ny);
Phi   = zeros(ny*Np, 1);
for i = 1:Np
    ri = (i-1)*ny + (1:ny);
    Gamma(ri,:) = C * Apow(i*ny + (1:ny), :);
    acc = zeros(ny,1);
    for m = 0:i-1, acc = acc + Apow(m*ny + (1:ny), :)*fd; end
    Phi(ri) = C * acc;
end

S = eye(nu*Np);
for i = 2:Np
    ri = (i-1)*nu + (1:nu);
    rj = (i-2)*nu + (1:nu);
    S(ri,rj) = -eye(nu);
end
E = [eye(nu); zeros(nu*(Np-1), nu)];
lambda_eff = max(lambda_fsw, 1e-6);
Lambdafsw_SE = lambda_eff * (S.'*E);
Lambdafsw_Ssquare =  lambda_eff*(S.'*S);


end

function Bs_TI = switch_to_alphabeta(Vdc)
Msw = eye(3) - ones(3)/3;
Tc  = (2/3) * [ 1, -1/2,      -1/2;
    0,  sqrt(3)/2, -sqrt(3)/2 ];   % Clarke (2x3)

Bs_TI = Tc * Vdc * Msw;                % 2x3

end

== matlab function FCSMPC_IdealSDA/FCS_MPC/BuildModel/BuildModel/Discretize_PMSM ==
  data: Bd output size=[2 2]; Ld input; Ad output size=[2 2]; Lq input; Rs input; Psi input; wel input; fd output size=[2 1]; Ts input
function [Bd, Ad, fd] = Discretize_PMSM(Ld, Lq, Rs, Psi, wel, Ts)

Ac = [ -Rs/Ld,        wel*Lq/Ld;
       -wel*Ld/Lq,  -Rs/Lq ];

Bc = [ 1/Ld, 0;
       0,    1/Lq ];

fc = [ 0;
      -wel*Psi/Lq ];

% Augmented matrix: states (2) + voltage inputs (2) + affine (1) = 5
M = [ Ac, Bc, fc;
      zeros(3,5) ];

Md = expm(M * Ts);

Ad   = Md(1:2, 1:2);
Bd = Md(1:2, 3:4);     % maps v_dq -> state increment
fd   = Md(1:2, 5);     % back-EMF contribution per step

== matlab function FCSMPC_IdealSDA/FCS_MPC/SDA_Solve/SDA Solve/Assembly_QP ==
  data: Ad input; Bd input; fd input; H output size=[3*Np 3*Np]; Gamma input; U_unc output size=[3*Np 1]; Phi input; Apow input; Lambdafsw_Ssquare input; Lambdafsw_SE input; Bs_TI input; idiq_fb input; idiq_ref input; theta_el input; wel input; Ts input; uprev input
function [H, U_unc] = fcn(Ad, Bd, fd, Gamma, Phi, Apow, ...
                          Lambdafsw_Ssquare, Lambdafsw_SE, Bs_TI, ...
                          idiq_fb, idiq_ref, theta_el, wel, Ts, uprev)
Np = 5;
nu = 3;  ny = 2;
% --- Schaltmatrizen: l = 0 fuer die Totzeit, l = 1..Np fuer den Horizont
Bs = zeros(ny, nu, Np+1);
for l = 0:Np
    th = theta_el + wel*Ts*l;
    Rp = [ cos(th), sin(th); -sin(th), cos(th) ];
    Bs(:,:,l+1) = Bd * Rp * Bs_TI;
end

% --- Totzeitkompensation: uprev wirkt im Intervall k -> k+1
idiq_k1 = Ad*idiq_fb + Bs(:,:,1)*uprev + fd;

% --- Praediktion ab k+1: U(j) wirkt im Intervall k+j -> k+j+1
Upsil = zeros(ny*Np, nu*Np);
for i = 1:Np
    ri = (i-1)*ny + (1:ny);
    for j = 1:i
        cj = (j-1)*nu + (1:nu);
        Upsil(ri,cj) = Apow((i-j)*ny + (1:ny), :) * Bs(:,:,j+1);
    end
end

W = Upsil.'*Upsil + Lambdafsw_Ssquare;

% --- Reverse Cholesky
n  = size(W,1);
Jx = fliplr(eye(n));
[Rt, p] = chol(Jx*W*Jx);
if p > 0
    Rt = eye(n);
end
H = Jx*Rt*Jx;

% --- lineare Terme
r = Gamma*idiq_k1 + Phi - repmat(idiq_ref, Np, 1);
F = Upsil.'*r - Lambdafsw_SE*uprev;

y     = H.' \ (-F);
U_unc = H   \ y;
end

== matlab function FCSMPC_IdealSDA/FCS_MPC/SDA_Solve/SDA Solve/SDA_Solve ==
  data: Jopt output; nodes output; optimal output; H input; U_unc input; NmaxNod input; Uopt output size=[3*Np 1]; Uapply output size=[3]; UoptPrev input
function [Jopt, nodes, optimal, Uopt, Uapply] = SDA_Solve(H, U_unc, NmaxNod, UoptPrev)
nu = 3;
V  = [0 1];
n  = numel(U_unc);
MAXIT = 100000;         % harte Obergrenze der Schleifendurchlaeufe

H     = double(H);
U_unc = double(U_unc);
Nmax  = double(NmaxNod);
Uprev = double(UoptPrev);
Ubar = H * U_unc;

Uround  = min(max(round(U_unc), V(1)), V(2));
Jround    = sum((H*(Uround - U_unc)).^2);

Ushift               = zeros(n,1);
Ushift(1:n-nu)       = Uprev(nu+1:n);
Ushift(n-nu+1:n)     = Uprev(n-nu+1:n);
Jshift               = sum((H*(Ushift - U_unc)).^2);

% --- den besseren als Inkumbente
if Jshift < Jround
    best = Jshift;
    Uopt = Ushift;
else
    best = Jround;
    Uopt = Uround;
end
nodes   = 0;
optimal = true;

U     = zeros(n,1);
d2s   = zeros(n+1,1);
cand  = zeros(n,2);
kidx  = zeros(n,1);
baseS = zeros(n,1);

i        = 1;
newLevel = true;

for it = 1:MAXIT
    if it >= MAXIT
        optimal = false;
    end
    ii = min(max(i,1), n);          % dem Coder die Schranke zeigen

    if newLevel
        acc = 0;
        for j = 1:n
            if j <= ii-1
                acc = acc + H(ii,j)*U(j);
            end
        end
        baseS(ii) = Ubar(ii) - acc;
        if baseS(ii) <= 0.5*H(ii,ii)
            cand(ii,1) = V(1);  cand(ii,2) = V(2);
        else
            cand(ii,1) = V(2);  cand(ii,2) = V(1);
        end
        kidx(ii) = 1;
        newLevel = false;
    end

    if kidx(ii) > 2
        i = i - 1;
        if i >= 1
            kidx(i) = kidx(i) + 1;
        end
        continue;
    end

    v     = cand(ii, kidx(ii));
    nodes = nodes + 1;
    if Nmax > 0 && nodes > Nmax
        optimal = false;
        break;
    end

    U(ii) = v;
    inc   = (H(ii,ii)*v - baseS(ii))^2;
    tot   = d2s(ii) + inc;

    if tot < best
        if ii == n
            best     = tot;
            Uopt     = U;
            kidx(ii) = kidx(ii) + 1;
        else
            d2s(ii+1) = tot;
            i         = i + 1;
            newLevel  = true;
        end
    else
        kidx(ii) = 3;
    end
end

Jopt   = best;
Uapply = Uopt(1:nu);
end

== stateflow chart FCSMPC_IdealSDA/FCS_MPC/CurrentRefCalc/Current_RateLimiter/RateLimiter ==
  settings: updateMethod=DISCRETE  sampleTime=FOC.SampleTime.TsSpeed
  state IDLE
  state Rising
    entry:  y =  fi(y_prev +dT * R, 1, 32, 18);
    exit: y_prev = y;
  state Falling
    entry:  y = fi(y_prev+dT * F, 1, 32, 18);
    exit: y_prev = y;
  state Directpassage
    entry:  y = u;
    exit: y_prev = y;
  (default) -> IDLE
  IDLE -> (junction 22)
  (junction 22) -> Rising [order 1] : [(u-y_prev)/dT>=R]
  (junction 22) -> Falling [order 2] : [(u-y_prev)/dT<=F]
  Rising -> (junction 22)
  Falling -> (junction 22)
  Directpassage -> (junction 22)
  (junction 22) -> Directpassage [order 3] : [(u-y_prev)/dT<R && (u-y_prev)/dT>F]
  data: u input fixdt(1,32,18); R input fixdt(1,32,18); F input fixdt(1,32,18); dT constant fixdt(1,32,18) size=1 =FOC.SampleTime.TsSpeed; y output fixdt(1,32,18); y_prev local fixdt(1,32,18) =0

== stateflow chart FCSMPC_IdealSDA/FCS_MPC/CurrentRefCalc/Current_RateLimiter/RateLimiter1 ==
  settings: updateMethod=DISCRETE  sampleTime=FOC.SampleTime.TsSpeed
  state IDLE
  state Rising
    entry:  y =  fi(y_prev +dT * R, 1, 32, 18);
    exit: y_prev = y;
  state Falling
    entry:  y = fi(y_prev+dT * F, 1, 32, 18);
    exit: y_prev = y;
  state Directpassage
    entry:  y = u;
    exit: y_prev = y;
  (default) -> IDLE
  IDLE -> (junction 22)
  (junction 22) -> Rising [order 1] : [(u-y_prev)/dT>=R]
  (junction 22) -> Falling [order 2] : [(u-y_prev)/dT<=F]
  Rising -> (junction 22)
  Falling -> (junction 22)
  Directpassage -> (junction 22)
  (junction 22) -> Directpassage [order 3] : [(u-y_prev)/dT<R && (u-y_prev)/dT>F]
  data: u input fixdt(1,32,18); R input fixdt(1,32,18); F input fixdt(1,32,18); dT constant fixdt(1,32,18) size=1 =FOC.SampleTime.TsSpeed; y output fixdt(1,32,18); y_prev local fixdt(1,32,18) =0

== stateflow chart FCSMPC_IdealSDA/FCS_MPC/CurrentRefCalc/RateLimiter ==
  settings: updateMethod=DISCRETE  sampleTime=FOC.SampleTime.TsSpeed
  state IDLE
  state Rising
    entry:  y =  fi(y_prev +dT * R, 1, 32, 18);
    exit: y_prev = y;
  state Falling
    entry:  y = fi(y_prev+dT * F, 1, 32, 18);
    exit: y_prev = y;
  state Directpassage
    entry:  y = u;
    exit: y_prev = y;
  (default) -> IDLE
  IDLE -> (junction 22)
  (junction 22) -> Rising [order 1] : [(u-y_prev)/dT>=R]
  (junction 22) -> Falling [order 2] : [(u-y_prev)/dT<=F]
  Rising -> (junction 22)
  Falling -> (junction 22)
  Directpassage -> (junction 22)
  (junction 22) -> Directpassage [order 3] : [(u-y_prev)/dT<R && (u-y_prev)/dT>F]
  data: u input fixdt(1,32,18); R input fixdt(1,32,18); F input fixdt(1,32,18); dT constant fixdt(1,32,18) size=1 =FOC.SampleTime.TsSpeed; y output fixdt(1,32,18); y_prev local fixdt(1,32,18) =0

== stateflow chart FCSMPC_IdealSDA/Plant_PMSM_INV/RateLimiter ==
  settings: updateMethod=DISCRETE  sampleTime=FOC.SampleTime.TsSpeed
  state IDLE
  state Rising
    entry:  y = dT*R+y_prev;
    exit: y_prev = y;
  state Falling
    entry:  y = dT*F+y_prev;
    exit: y_prev = y;
  state Directpassage
    entry:  y = u;
    exit: y_prev = y;
  (default) -> IDLE
  IDLE -> (junction 22)
  (junction 22) -> Rising [order 1] : [(u-y_prev)/dT>=R]
  (junction 22) -> Falling [order 2] : [(u-y_prev)/dT<=F]
  Rising -> (junction 22)
  Falling -> (junction 22)
  Directpassage -> (junction 22)
  (junction 22) -> Directpassage [order 3] : [(u-y_prev)/dT<R && (u-y_prev)/dT>F]
  data: u input; R input; F input; dT constant double size=1 =FOC.SampleTime.TsSpeed; y output; y_prev local double =0
